simulink model "SD_Datalogger"  (Simulink 7.6)
settings: Solver=FixedStepDiscrete  SolverMode=SingleTasking  StartTime=0.0  StopTime=10.0  FixedStep=0.001  RelTol=1e-3
undefined symbols (not defined in the file or in its folder): FSclose, FSinit, FSprint, Init_onlyOnce, Init_Reset, u1
libraries: dsPICdrivers x14, simulink x1, dspswit3 x1
settings Model: Creator=konstantin.avdashche  LastModifiedBy=ij8977
settings OptimizationCC: OptimizeModelRefInitCode=on  LifeSpan=1
settings RTWCC: SystemTargetFile=pic32.tlc  MakeCommand=make_CreateMPLAB  TemplateMakefile=pic32_gcc.tmf  PostCodeGenCommand=dsPIC_Compile()  Description=Embedded Target for Microchip dsPIC (real-time)  ProcessScript=pic32_make_rtw_hook
settings RTWCC: CustomInclude=|
  | "C:\Users\ij8977\Documents\MatlabWork\SD_Datalogging"
  | "C:\Users\ij8977\Documents\MatlabWork\Microchip"
  | "C:\Users\ij8977\Documents\MatlabWork\Microchip\Include\MDD File System"
settings RTWCC: CustomSource=|
  | "C:\Users\ij8977\Documents\MatlabWork\SD_Datalogging\CustomSD.c"
  | "C:\Users\ij8977\Documents\MatlabWork\SD_Datalogging\SD-SPI.c"
  | "C:\Users\ij8977\Documents\MatlabWork\SD_Datalogging\FSIO.c"
settings CodeAppCC: IgnoreCustomStorageClasses=off
settings STFCustomTargetCC: IncludeMdlTerminateFcn=off  CombineOutputUpdateFcns=on  SuppressErrorStatus=on  ERTCustomFileBanners=on  SupportContinuousTime=off  SupportNonInlinedSFcns=off  SystemTargetFile=pic32.tlc
settings ERTTargetCC: MultiwordLength=2048  ParMdlRefBuildCompliant=off  CompOptLevelCompliant=off  IncludeMdlTerminateFcn=off  SuppressErrorStatus=on  ERTFirstTimeCompliant=off  ModelStepFunctionPrototypeControlCompliant=off  CPPClassGenCompliant=off  ExtModeMexFile=noextcomm  InlinedParameterPlacement=NonHierarchical  ERTSrcFileBannerTemplate=dsPIC_code_template.cgt  ERTHdrFileBannerTemplate=dsPIC_code_template.cgt  ERTDataSrcFileTemplate=dsPIC_code_template.cgt  ERTDataHdrFileTemplate=dsPIC_code_template.cgt  ERTCustomFileTemplate=dsPIC_main.tlc  ConvertIfToSwitch=off
settings CustomProperty: DataType=string  Value=C:\PROGRA~1\MATLAB\R2010B~1\bin\win32\gmake

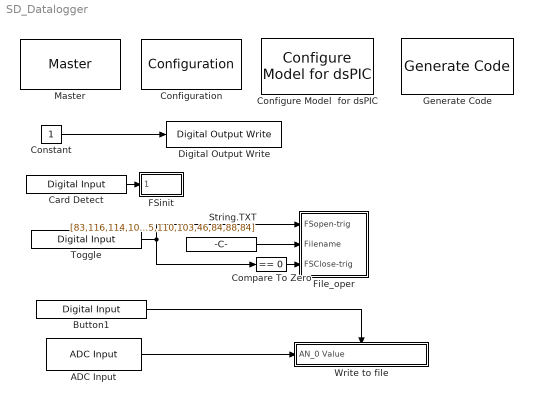
== system SD_Datalogger ==
  ADC Input : dsPICdrivers/Peripheral I//O/ADC Input  Tag=dsPIC_ADC  Priority=5  ADC_TYPE=10 bits  ADC_MODE=Continuous sampling & get last channel value  NbrSampleStep=1  VoltRefpopup="AVdd  -  AVss"  OutFormatBitspopup=0000 00dd dddd dddd : Integer  InterruptPriority=6  ANCHANNELS=[0]  MaxName=ANmax = 1023  Rin=1e2  ADCS=12  SAMC=1  Temperature=25  DMAChannel=0  SampleTime=-1  Status="OK  |  Tsmp=1.625e-007 |  T/Channel=2.113e-006 |  Tall=2.113e-006"  SSRC=auto convert
  Button1 : dsPICdrivers/Digital I//O/Digital Input  Tag=dsPIC_Digital_Input  PORT=A  Pin=[6]  SampleTime=-1  OrderingInOutPopup=None
  Card Detect : dsPICdrivers/Digital I//O/Digital Input  Tag=dsPIC_Digital_Input  PORT=D  Pin=[4]  SampleTime=-1  OrderingInOutPopup=None
  Compare To Zero : simulink/Logic and Bit Operations/Compare To Zero  SystemSampleTime=-1  relop===  LogicOutDataTypeMode=uint8
  Configuration : dsPICdrivers/Configuration  SystemSampleTime=-1  double64=on
  Configure Model  for dsPIC : dsPICdrivers/Simulink Configuration/Configure Model  for dsPIC
  Constant : Constant  OutDataTypeStr=Inherit: Inherit via back propagation
  Digital Output Write : dsPICdrivers/Digital I//O/Digital Output Write  Tag=dsPIC_Digital_Output  Priority=5  PORT=F  Pin=[2]  Simultaneous=off  OrderingInOutPopup=None
  FSinit : Subsystem  TreatAsAtomicUnit=on
  File_oper : Subsystem  TreatAsAtomicUnit=on
  Generate Code : dsPICdrivers/Simulink Configuration/Generate Code
  Master : dsPICdrivers/Master  Tag=dsPIC_MASTER  Priority=1  TimeStepType=Timer1  picType=32MX460F512L  fcy=40000000  Quartz_33f=8e6  PLLActive_33f=on  fcyDesired_33f=40e6  tmr1="[1  39999  0]"  tmr1Info="Time Step : 0.001  ;   Error : 0%  PR1=39999"  tmr2345="[0  0  0  0]"  tmr2345cfg=[-1 -1 -1 -1]  IOautoConf=on  typePort="[ 0   0   0   0   0   0   9   0   0   0   0   0   0   0   0   0   8   0   0   0   0   0   0   0   0   0  10   0   0   0   0   0   0   0   0   0   0   0   0   0   0   0   0   0   0   0   0   0   0   0   0   0   9   0   0   0   0   0   0   0   0   0   0   0   0   0   0   0   0   0   0   0   0   0   0   0   0   0   0   0   0   0  10   0   0   0   0   0   9   0   0   0   0   0   0   0   0   0   0   0   0   0   0   0   0   0   0   0   0   0   0   0 ]"  TRIS="[ 65535  64511  65535  65535  65535  65531  65535 ]"  ADPCFG=1024  MasterBusyPort=None  MasterOverloadPort=None  FOSC=Quartz (XT - HS)  ClockSwitchMonitor=Both disabled  TempProtection_33f=TEMP_ON  FPBOR=<empty>  PWRT=disable  MCLR=<empty>  ICD=ICS_PGD1  JTAGEN=JTAGEN_OFF  PowerSave=off  OverrideFcy=off  NewFcy=1e6  PR2345="[65535  65535  65535  65535]"
  String.TXT : Constant  Value=[83,116,114,105,110,103,46,84,88,84]  OutDataTypeStr=uint8
  Toggle : dsPICdrivers/Digital I//O/Digital Input  Tag=dsPIC_Digital_Input  PORT=F  Pin=[8]  SampleTime=-1  OrderingInOutPopup=None
  Write to file : Subsystem  TreatAsAtomicUnit=on
  wires:
  String.TXT/1 -> File_oper/2(Filename)
  Card Detect/1 -> FSinit/1(Card_in)
  Constant/1 -> Digital Output Write/1
  Compare To Zero/1 -> File_oper/3(FSClose-trig)
  Toggle/1 -> Compare To Zero/1, File_oper/1(FSopen-trig)
  ADC Input/1 -> Write to file/1(AN_0 Value)
  Button1/1 -> Write to file/Trigger

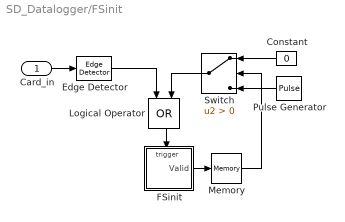
== system SD_Datalogger/FSinit ==
  Card_in : Inport
  Constant : Constant  Value=0
  Edge Detector : dspswit3/Edge Detector  SystemSampleTime=-1  InputProcessing=Inherited (this choice will be removed - see release notes)
  FSinit : Subsystem  TreatAsAtomicUnit=on
  Logical Operator : Logic  Operator=OR  AllPortsSameDT=off  OutDataTypeStr=boolean
  Memory : Memory
  Pulse Generator : DiscretePulseGenerator  PulseWidth=2  SampleTime=-1
  Switch : Switch  Criteria=u2 > Threshold
  wires:
  Card_in/1 -> Edge Detector/1
  Edge Detector/1 -> Logical Operator/1
  Switch/1 -> Logical Operator/2
  Logical Operator/1 -> FSinit/Trigger
  Constant/1 -> Switch/1
  Pulse Generator/1 -> Switch/3
  FSinit/1(Valid) -> Memory/1
  Memory/1 -> Switch/2

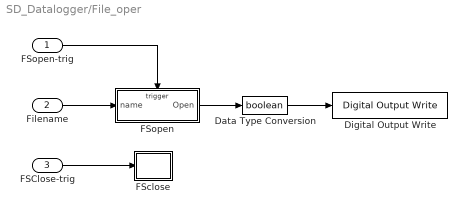
== system SD_Datalogger/File_oper ==
  FSopen-trig : Inport
  Filename : Inport  Port=2
  FSClose-trig : Inport  Port=3
  Data Type Conversion : DataTypeConversion  OutDataTypeStr=boolean
  Digital Output Write : dsPICdrivers/Digital I//O/Digital Output Write  Tag=dsPIC_Digital_Output  Priority=5  PORT=B  Pin=[10]  Simultaneous=off  OrderingInOutPopup=None
  FSclose : Subsystem  TreatAsAtomicUnit=on
  FSopen : Subsystem  TreatAsAtomicUnit=on
  wires:
  Filename/1 -> FSopen/1(name)
  FSopen-trig/1 -> FSopen/Trigger
  FSopen/1(Open) -> Data Type Conversion/1
  FSClose-trig/1 -> FSclose/Trigger
  Data Type Conversion/1 -> Digital Output Write/1

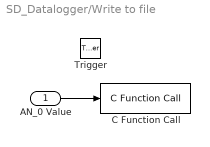
== system SD_Datalogger/Write to file ==
  AN_0 Value : Inport
  Trigger : TriggerPort
  C Function Call : dsPICdrivers/OTHERS/C Function Call  Tag=dsPIC_dsPIC_CFunctionCall  FctUpdate=Output Function  fctName='FSprint'  INPUT_SIZE=1  INPUT1=uint16  INPUT2=--  INPUT3=--  OUTPUT_SIZE=1  OUTPUT1=--  SampleTime=-1  InputType=[ 4 ]  OutputType=[ ]  FctDeclaration=extern void FSprint(uint16_T u1);  FctCall=FSprint(%u1);  OrderingInOutPopup=None  FctStart=None  FctStart_Name=Init_onlyOnce  FctStart_Declaration=inline extern void Init_onlyOnce();  FctStart_Call=Init_onlyOnce();  FctInit=None  FctInit_Name=Init_Reset  FctInit_Declaration=inline extern void Init_Reset();  FctInit_Call=Init_Reset();
  wires:
  AN_0 Value/1 -> C Function Call/1

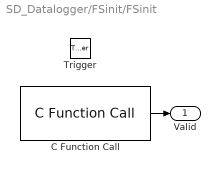
== system SD_Datalogger/FSinit/FSinit ==
  Trigger : TriggerPort
  C Function Call : dsPICdrivers/OTHERS/C Function Call  Tag=dsPIC_dsPIC_CFunctionCall  FctUpdate=Output Function  fctName='FS_init_loop'  INPUT_SIZE=0  INPUT1=--  INPUT2=--  INPUT3=--  OUTPUT_SIZE=1  OUTPUT1=uint8  SampleTime=-1  InputType=[ ]  OutputType=[ 2 ]  FctDeclaration=extern uint8_T FS_init_loop();  FctCall=%y1 = FS_init_loop();  OrderingInOutPopup=None  FctStart=None  FctStart_Name=Init_onlyOnce  FctStart_Declaration=inline extern void Init_onlyOnce();  FctStart_Call=Init_onlyOnce();  FctInit=None  FctInit_Name=FSinit  FctInit_Declaration=inline extern void FSinit();  FctInit_Call=FSinit();
  Valid : Outport
  wires:
  C Function Call/1 -> Valid/1

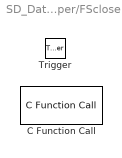
== system SD_Datalogger/File_oper/FSclose ==
  Trigger : TriggerPort
  C Function Call : dsPICdrivers/OTHERS/C Function Call  Tag=dsPIC_dsPIC_CFunctionCall  FctUpdate=Output Function  fctName='FSclose'  INPUT_SIZE=1  INPUT1=--  INPUT2=--  INPUT3=--  OUTPUT_SIZE=1  OUTPUT1=--  SampleTime=-1  InputType=[ ]  OutputType=[ ]  FctDeclaration=extern void FSclose();  FctCall=FSclose();  OrderingInOutPopup=None  FctStart=None  FctStart_Name=Init_onlyOnce  FctStart_Declaration=inline extern void Init_onlyOnce();  FctStart_Call=Init_onlyOnce();  FctInit=None  FctInit_Name=Init_Reset  FctInit_Declaration=inline extern void Init_Reset();  FctInit_Call=Init_Reset();

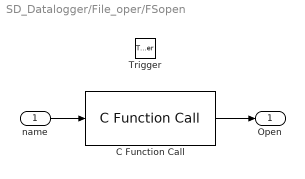
== system SD_Datalogger/File_oper/FSopen ==
  name : Inport
  Trigger : TriggerPort
  C Function Call : dsPICdrivers/OTHERS/C Function Call  Tag=dsPIC_dsPIC_CFunctionCall  FctUpdate=Output Function  fctName='FSopen'  INPUT_SIZE=10  INPUT1=uint8  INPUT2=--  INPUT3=--  OUTPUT_SIZE=1  OUTPUT1=int16  SampleTime=-1  InputType=[ 2 ]  OutputType=[ 3 ]  FctDeclaration=extern int16_T FSopen(uint8_T* u1);  FctCall=%y1 = FSopen(*%u1);  OrderingInOutPopup=None  FctStart=None  FctStart_Name=Init_onlyOnce  FctStart_Declaration=inline extern void Init_onlyOnce();  FctStart_Call=Init_onlyOnce();  FctInit=None  FctInit_Name=Init_Reset  FctInit_Declaration=inline extern void Init_Reset();  FctInit_Call=Init_Reset();
  Open : Outport
  wires:
  name/1 -> C Function Call/1
  C Function Call/1 -> Open/1
